simulink model "decodeur_hamming"  (R2023b)
settings: Solver=FixedStepDiscrete  StartTime=0.0  StopTime=10.0  FixedStep=Tc_reg  RelTol=1e-3
libraries: simulink x7
settings Model: Creator=e2405714  LastModifiedBy=e2405714

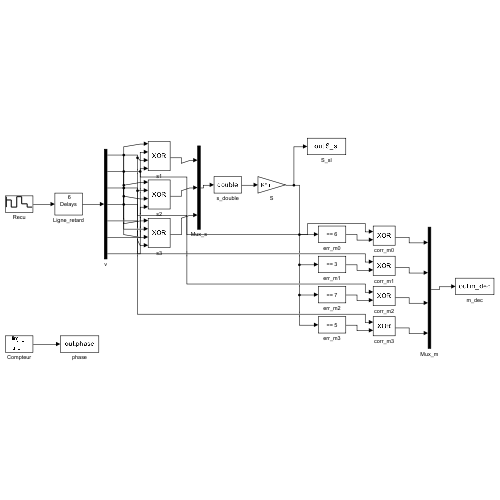
[thumbnail: Simulink's stored preview of the top-level diagram]
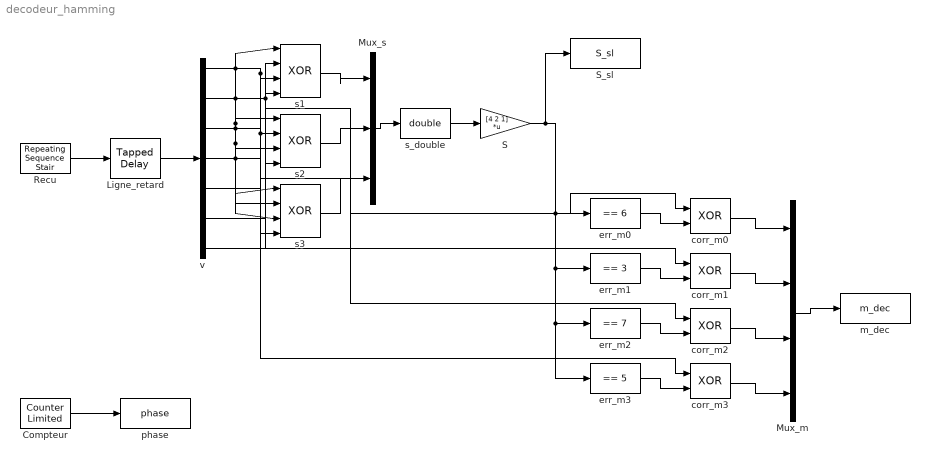
== system decodeur_hamming ==
  Compteur : simulink/Sources/Counter Limited  uplimit=6  tsamp=Tc_reg
  Ligne_retard : simulink/Discrete/Tapped Delay  vinit=0  samptime=Tc_reg  NumDelays=6  DelayOrder=Oldest  includeCurrent=on
  Mux_m : Mux
  Mux_s : Mux  Inputs=3
  Recu : simulink/Sources/Repeating Sequence Stair  OutValues=seq_rx  tsamp=Tc_reg  OutMin=[]  OutMax=[]  OutDataTypeStr=double  OutputDataTypeScalingMode=double  OutDataType=fixdt(0,8)  ConRadixGroup=Best Precision: Vector-wise  OutScaling=2^-12
  S : Gain  Gain=[4 2 1]  Multiplication=Matrix(K*u)
  S_sl : ToWorkspace  VariableName=S_sl  SampleTime=-1
  corr_m{0..3} (4 alike) : Logic  Operator=XOR  AllPortsSameDT=off  OutDataTypeStr=boolean
  err_m0 : simulink/Logic and Bit Operations/Compare To Constant  relop===  const=6  OutDataTypeStr=boolean
  err_m1 : simulink/Logic and Bit Operations/Compare To Constant  relop===  const=3  OutDataTypeStr=boolean
  err_m2 : simulink/Logic and Bit Operations/Compare To Constant  relop===  const=7  OutDataTypeStr=boolean
  err_m3 : simulink/Logic and Bit Operations/Compare To Constant  relop===  const=5  OutDataTypeStr=boolean
  m_dec : ToWorkspace  VariableName=m_dec  SampleTime=-1
  phase : ToWorkspace  VariableName=phase  SampleTime=-1
  s1 : Logic  Operator=XOR  Inputs=4  AllPortsSameDT=off  OutDataTypeStr=boolean
  s2 : Logic  Operator=XOR  Inputs=4  AllPortsSameDT=off  OutDataTypeStr=boolean
  s3 : Logic  Operator=XOR  Inputs=4  AllPortsSameDT=off  OutDataTypeStr=boolean
  s_double : DataTypeConversion  OutDataTypeStr=double  SaturateOnIntegerOverflow=off  RndMeth=Floor
  v : Demux  Outputs=7
  wires:
  Compteur/1 -> phase/1
  Recu/1 -> Ligne_retard/1
  Ligne_retard/1 -> v/1
  v/4 -> s1/1, s2/1, corr_m0/1
  v/2 -> s2/3, s3/2, s1/2, corr_m2/1
  v/1 -> s1/3, corr_m3/1, s3/3
  v/7 -> s1/4
  v/3 -> s2/2, corr_m1/1, s3/1
  v/6 -> s2/4
  v/5 -> s3/4
  s1/1 -> Mux_s/1
  s2/1 -> Mux_s/2
  s3/1 -> Mux_s/3
  Mux_s/1 -> s_double/1
  s_double/1 -> S/1
  S/1 -> err_m2/1, err_m3/1, err_m1/1, err_m0/1, S_sl/1
  err_m0/1 -> corr_m0/2
  corr_m0/1 -> Mux_m/1
  err_m1/1 -> corr_m1/2
  corr_m1/1 -> Mux_m/2
  err_m2/1 -> corr_m2/2
  corr_m2/1 -> Mux_m/3
  err_m3/1 -> corr_m3/2
  corr_m3/1 -> Mux_m/4
  Mux_m/1 -> m_dec/1
